simulink model "Controller_damping_cbf_22"  (R2022b)
settings: Solver=ode4  StartTime=0.0  StopTime=Inf  FixedStep=1e-3  RelTol=1e-3
values from neighbouring files (symbols this model uses):
  cbf_damping_params = [cbf_p_ths; cbf_v_ths; cbf_v_0; cbf_gamma; cbf_d_max;                        cbf_w_lin; cbf_w_quad; plane_normal; plane_offset;                        cbf_latch_entry; cbf_zone_hyst; cbf_latch_alpha; cbf_clip_drift;                        cbf_tau_rate; cbf_dt; cbf_gamma_pos_scale]    [init_damping_cbf.m]
  Dn = 20 * ones(7,1)    [init_damping_cbf.m]
  H_0_cy = H_0_pr * H_pr_cy    [init_damping_cbf.m]
  H_home = getTransform(Franka_robot, q_home, 'panda_link8', 'panda_link0')    [init_damping_cbf.m]
  Kn = 0 * ones(7,1)    [init_damping_cbf.m]
  q_home = q_init    [init_damping_cbf.m]
  q_init = [0 0  0  -(2/4)*pi  0  pi/2  -pi/4]'    [init_damping_cbf.m]
undefined symbols (not defined in the file or in its folder): DiscIntNeverNeededParam, Fext_mag, T_final, X, Y, Z
libraries: sm_lib x162, nesl_utility x44, matrix_library x3, Robotics_lib x1
(part 1 of 12)
settings Model: Creator=nthelenb  LastModifiedBy=galileo
settings ConfigComp: CovMetricSettings=de  CovBoundaryAbsTol=1.0e-5
settings SimscapeCC: SimscapeUseEnergyAccounting=off

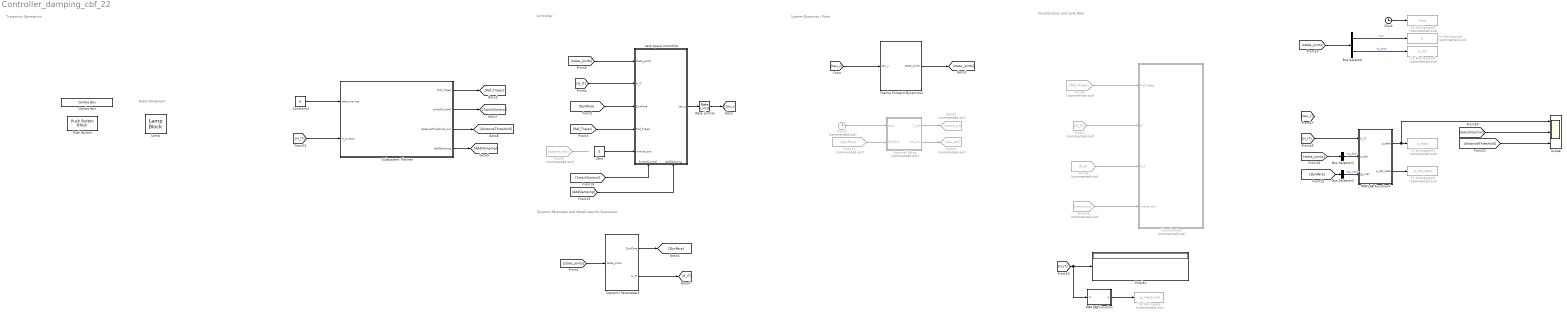
== system Controller_damping_cbf_22 ==
  note: Visualiszation and save Data
  note: Robot Movement
  note: Dynamic Parameter and Model Specific Quantities
  note: System Dynamics / Plant
  note: Trajectory Generation
  note: Controller
  Bus Selector : BusSelector  OutputSignals=q,q_dot
  Bus Selector1 : BusSelector  OutputSignals=q_dot
  Bus Selector2 : BusSelector  OutputSignals=Jg_mat
  Clock : Clock
  Clock1 : Clock  Commented=on
  Combo Box : ComboBox  LabelPosition=Hide  SelectedLabel=Move Gravi. Comp
      settings: Values={{'Go Home', 'Move Gravi. Comp', 'Move Add Damp'}, [1 2 3]}
  Constant3 : Constant  Value=0
  Display : Display
  Dynamic Parameters : Subsystem
  External Force : Subsystem  Commented=on
  Franka Forward Dynamics2 : Subsystem
  From11 : From  Commented=on  GotoTag=DynPara
  From14 : From  Commented=on  GotoTag=wrench_ext
  From5 : From  Commented=on  GotoTag=K_d
  From7 : From  Commented=on  GotoTag=H_IT
  From8 : From  Commented=on  GotoTag=Ref_Trajec
  From9 : From  Commented=on  GotoTag=wrench_ext
  Goto5 : Goto  Commented=on  GotoTag=wrench_ext
  Goto6 : Goto  Commented=on  GotoTag=tau_ext
  Lamp : LampBlock  LabelPosition=Hide
  MATLAB Function : MATLAB Function  TreatAsAtomicUnit=on
  MATLAB Function4 : MATLAB Function  TreatAsAtomicUnit=on
  Push Button : PushButtonBlock  ButtonText=Move Robot  OffValue=0.000000
  Rate Limiter : RateLimiter  RisingSlewLimit=999  FallingSlewLimit=-999  SampleTimeMode=inherited
  Scope : Scope  NumInputPorts=3
  Subsystem: Planner : Subsystem
  To Workspace : ToWorkspace  Commented=on  VariableName=p_measured  SampleTime=-1
  To Workspace3 : ToWorkspace  Commented=on  VariableName=q  SampleTime=-1
  To Workspace4 : ToWorkspace  Commented=on  VariableName=q_dot  SampleTime=-1
  To Workspace5 : ToWorkspace  Commented=on  VariableName=p_data  SampleTime=-1
  To Workspace6 : ToWorkspace  Commented=on  VariableName=p_dot_data  SampleTime=-1
  To Workspace8 : ToWorkspace  Commented=on  VariableName=time  SampleTime=-1
  Visualisation : Subsystem  Commented=on
  Zero : Constant  Value=0  OutDataTypeStr=Inherit: Inherit via back propagation
  task space controller : Subsystem
      settings: PortSchema="{\"entries\":[{\"content\":{\"sides\":[{\"content\":{\"connectorIds\":[\"In1\",\"In2\",\"In3\",\"In4\",\"In5\"]},\"type\":\"ConnectorPlacement.EquallySpacedRectSide\",\"uuid\":\"77049308-6373-4cc5-ac04-ffe2481fe586\"},{\"content\":{\"connectorIds\":[\"Out1\"],\"side\":\"RIGHT\"},\"type\":\"ConnectorPlacement.EquallySpacedRectSide\",\"uuid\":\"f03c39fe-2f04-4b7b-9f47-c34b5694c009\"},{\"content\":{\"connectorIds\":[],\"side\":\"TOP\"},\"type\":\"ConnectorPlacement.EquallySpacedRectSide\",\"uuid\":\"88522150-2a14-460b-940a-8c2ff3633826\"},{\"content\":{\"connectorIds\":[\"In6\",\"In7\"],\"side\":\"BOTTOM\"},\"type\":\"ConnectorPlacement.EquallySpacedRectSide\",\"uuid\":\"dd94313b-0570-425b-8d26-1c571736a013\"}]},\"type\":\"ConnectorPlacement.EquallySpacedConnector\",\"uuid\":\"5aa11ebf-be9b-4d28-87ba-ea9d43661d80\"}],\"packageUris\":[\"http://schema.mathworks.com/mf0/Connector/R2020b\"],\"version\":\"1.0\"}"
  wires:
  External Force/1(F_ext) -> Goto5/1
  From11/1 -> External Force/2(DynPara)
  Clock1/1 -> External Force/1(time)
  External Force/2(tau_ext) -> Goto6/1
  Franka Forward Dynamics2/1(state_joints) -> [state_joints]
  [tau_c] -> Franka Forward Dynamics2/1(tau_c)
  [state_joints] -> Dynamic Parameters/1(state_joints)
  Zero/1 -> task space controller/5(wrench_ext)
  From7/1 -> Visualisation/2(H)
  [AddDamping] -> task space controller/7(AddDamping)
  Subsystem: Planner/4(AddDamping) -> [AddDamping]
  Clock/1 -> To Workspace8/1
  Constant3/1 -> Subsystem: Planner/1(start_moving)
  Bus Selector2/1 -> MATLAB Function4/3(Jg_mat)  "<Jg_mat>"
  [distanceThreshold] -> Scope/3
  [H_IT] -> task space controller/2(H_IT)
  From9/1 -> ?
  From8/1 -> Visualisation/1(Ref_Trajec)
  [state_joints] -> task space controller/1(state_joints)
  Subsystem: Planner/3(distanceThreshold_out) -> [distanceThreshold]
  MATLAB Function4/1(p_data) -> Scope/1, To Workspace5/1
  From14/1 -> Visualisation/4(wrench_ext)
  [SwitchControl] -> Scope/2
  [DynPara] -> Bus Selector2/1
  Bus Selector/2 -> To Workspace4/1  "<q_dot>"
  [SwitchControl] -> task space controller/6(SwitchControl)
  MATLAB Function4/2(p_dot_data) -> To Workspace6/1
  Subsystem: Planner/1(Ref_Trajec) -> [Ref_Trajec]
  [state_joints] -> Bus Selector/1
  [state_joints] -> Bus Selector1/1
  Subsystem: Planner/2(switchControl) -> [SwitchControl]
  [H_IT] -> MATLAB Function4/1(H_IT)
  Rate Limiter/1 -> [tau_c]
  Bus Selector1/1 -> MATLAB Function4/2(q_dot)  "<q_dot>"
  task space controller/1(tau_c) -> Rate Limiter/1
  [H_IT] -> MATLAB Function/1(H), Display/1
  [Ref_Trajec] -> task space controller/4(Ref_Trajec)
  [DynPara] -> task space controller/3(DynPara)
  MATLAB Function/1(p) -> To Workspace/1
  Dynamic Parameters/1(DynPara) -> [DynPara]
  Bus Selector/1 -> To Workspace3/1  "<q>"
  [H_IT] -> Subsystem: Planner/2(H_current)
  From5/1 -> Visualisation/3(K_d)
  Dynamic Parameters/2(H_IT) -> [H_IT]

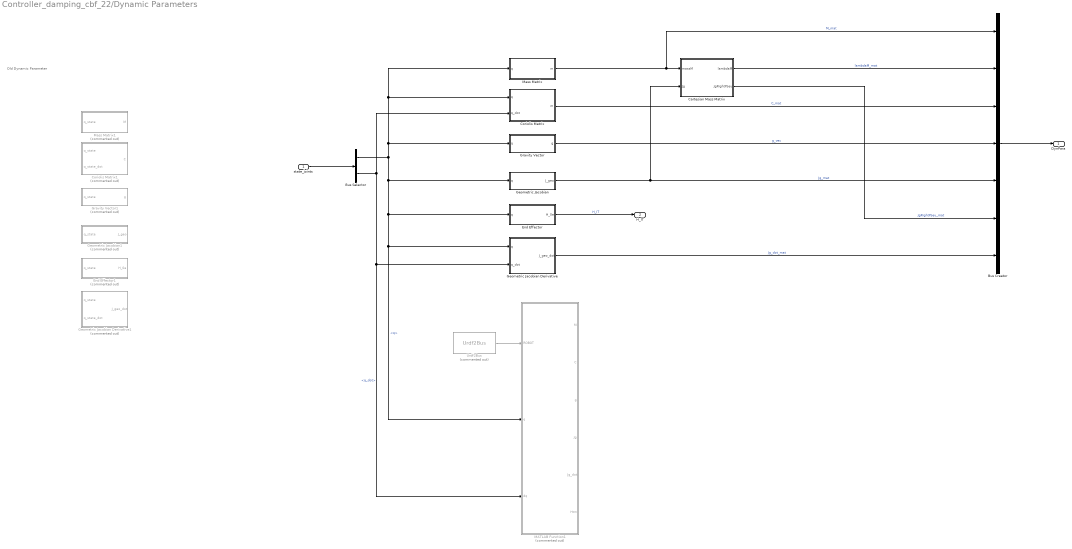
== system Controller_damping_cbf_22/Dynamic Parameters ==
  note: Old Dynamic Parameter
  state_joints : Inport
  Bus Creator : BusCreator  Inputs=7
  Bus Selector : BusSelector  OutputSignals=q,q_dot
  Cartesian Mass Matrix : MATLAB Function  TreatAsAtomicUnit=on
  Coriolis Matrix : MATLAB Function  TreatAsAtomicUnit=on
  Coriolis Matrix1 : MATLAB Function  Commented=on  TreatAsAtomicUnit=on
  End Effector : MATLAB Function  TreatAsAtomicUnit=on
  End Effector1 : MATLAB Function  Commented=on  TreatAsAtomicUnit=on
  Geometric Jacobian : MATLAB Function  TreatAsAtomicUnit=on
  Geometric Jacobian Derivative : MATLAB Function  TreatAsAtomicUnit=on
  Geometric Jacobian Derivative1 : MATLAB Function  Commented=on  TreatAsAtomicUnit=on
  Geometric Jacobian1 : MATLAB Function  Commented=on  TreatAsAtomicUnit=on
  Gravity Vector : MATLAB Function  TreatAsAtomicUnit=on
  Gravity Vector1 : MATLAB Function  Commented=on  TreatAsAtomicUnit=on
  MATLAB Function1 : MATLAB Function  Commented=on  TreatAsAtomicUnit=on
  Mass Matrix : MATLAB Function  TreatAsAtomicUnit=on
  Mass Matrix1 : MATLAB Function  Commented=on  TreatAsAtomicUnit=on
  Urdf2Bus : Robotics_lib/Urdf2Bus  Commented=on  filename='Franka_arm.urdf'  tcp=9  S=[]
  DynPara : Outport
  H_IT : Outport  Port=2
  wires:
  state_joints/1 -> Bus Selector/1
  Urdf2Bus/1 -> MATLAB Function1/1(ROBOT)
  Bus Selector/1 -> Coriolis Matrix/1(q), Mass Matrix/1(q), Gravity Vector/1(q), Geometric Jacobian/1(q), MATLAB Function1/2(q), Geometric Jacobian Derivative/1(q), End Effector/1(q)  "<q>"
  Bus Selector/2 -> Geometric Jacobian Derivative/2(q_dot), MATLAB Function1/3(dq), Coriolis Matrix/2(q_dot)  "<q_dot>"
  Mass Matrix/1(m) -> Bus Creator/1, Cartesian Mass Matrix/1(massM)  "M_mat"
  Bus Creator/1 -> DynPara/1
  Cartesian Mass Matrix/1(lambdaM) -> Bus Creator/2  "lambdaM_mat"
  Coriolis Matrix/1(m) -> Bus Creator/3  "C_mat"
  Gravity Vector/1(g) -> Bus Creator/4  "g_vec"
  Cartesian Mass Matrix/2(JgRightPseu) -> Bus Creator/6  "JgRightPseu_mat"
  Geometric Jacobian Derivative/1(J_geo_dot) -> Bus Creator/7  "Jg_dot_mat"
  End Effector/1(H_0e) -> H_IT/1  "H_IT"
  Geometric Jacobian/1(J_geo) -> Cartesian Mass Matrix/2(Jg), Bus Creator/5  "Jg_mat"

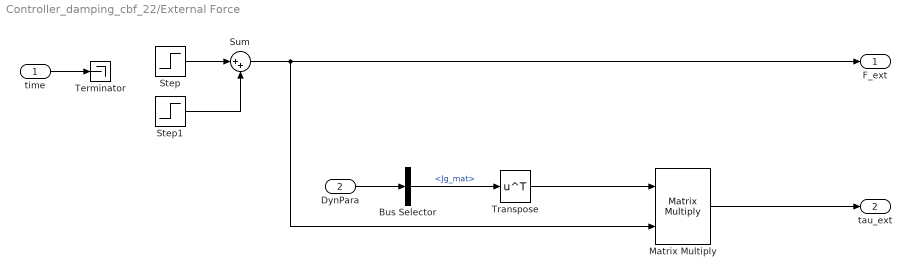
== system Controller_damping_cbf_22/External Force ==
  time : Inport
  DynPara : Inport  Port=2
  Bus Selector : BusSelector  OutputSignals=Jg_mat
  Matrix Multiply : Product  Multiplication=Matrix(*)
  Step : Step  Time=5  Before=zeros(6,1)  After=Fext_mag.*[1;zeros(5,1)]  SampleTime=0
  Step1 : Step  Time=12  Before=zeros(6,1)  After=-Fext_mag.*[1;zeros(5,1)]  SampleTime=0
  Sum : Sum  Inputs=|++
  Terminator : Terminator
  Transpose : Math  Operator=transpose
  F_ext : Outport
  tau_ext : Outport  Port=2
  wires:
  Step/1 -> Sum/1
  Step1/1 -> Sum/2
  time/1 -> Terminator/1
  Sum/1 -> Matrix Multiply/2, F_ext/1
  Transpose/1 -> Matrix Multiply/1
  Bus Selector/1 -> Transpose/1  "<Jg_mat>"
  DynPara/1 -> Bus Selector/1
  Matrix Multiply/1 -> tau_ext/1

== system Controller_damping_cbf_22/Franka Forward Dynamics2 ==
  note: NO joint Limits
  note: With joint Limits
  tau_c : Inport
  Bus Creator : BusCreator  Inputs=2
  Franka Forward Dynamics [SimMechanics] : Subsystem
  Franka Forward Dynamics [SimMechanics]1 : Subsystem  Commented=on
  state_joints : Outport
  wires:
  Franka Forward Dynamics [SimMechanics]/1(q) -> Bus Creator/1  "q"
  Franka Forward Dynamics [SimMechanics]/2(q_dot) -> Bus Creator/2  "q_dot"
  tau_c/1 -> Franka Forward Dynamics [SimMechanics]/1(tau)
  Bus Creator/1 -> state_joints/1

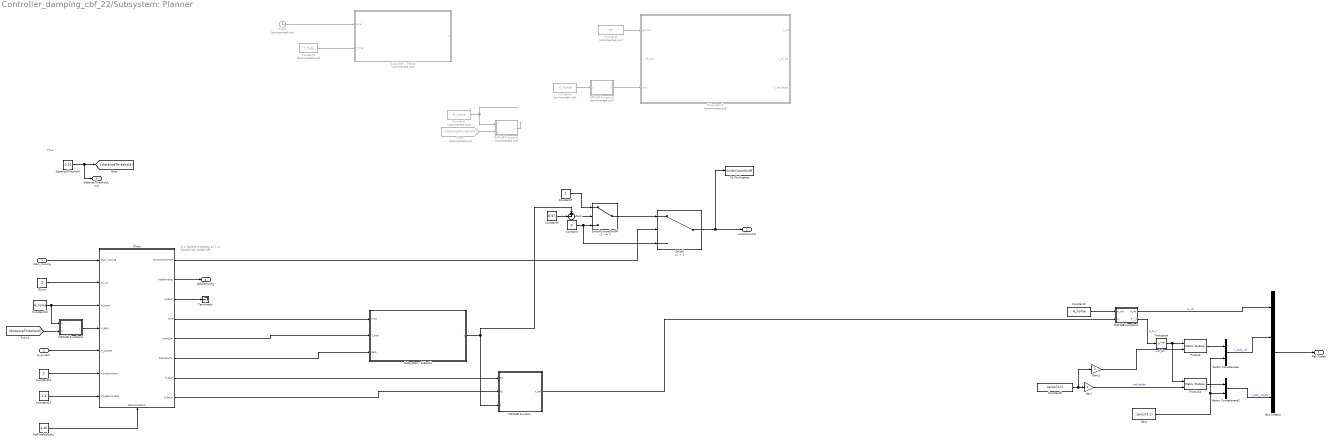
== system Controller_damping_cbf_22/Subsystem: Planner ==
  note: 0 = Control is always on
      | 1 = Control can switch off
  note: Para
  start_moving : Inport
  H_current : Inport  Port=2
  Bus Creator : BusCreator  Inputs=4
  Chart : Stateflow chart  TreatAsAtomicUnit=on
      settings: PortSchema="{\"entries\":[{\"content\":{\"sides\":[{\"content\":{\"connectorIds\":[\"In2\",\"In3\",\"In5\",\"In4\",\"In6\",\"In7\",\"In8\"]},\"type\":\"ConnectorPlacement.EquallySpacedRectSide\",\"uuid\":\"9d0e544c-68a3-4d0d-81a9-b4a9e24909b9\"},{\"content\":{\"connectorIds\":[\"Out1\",\"Out2\",\"Out4\",\"Out5\",\"Out3\",\"Out6\",\"Out7\",\"Out8\"],\"side\":\"RIGHT\"},\"type\":\"ConnectorPlacement.EquallySpacedRectSide\",\"uuid\":\"6b3881b7-7b6b-4877-af69-7085981ee4af\"},{\"content\":{\"connectorIds\":[],\"side\":\"TOP\"},\"type\":\"ConnectorPlacement.EquallySpacedRectSide\",\"uuid\":\"e07b297f-72d7-4e07-a8ff-78e8d5f0a2d3\"},{\"content\":{\"connectorIds\":[\"In1\"],\"side\":\"BOTTOM\"},\"type\":\"ConnectorPlacement.EquallySpacedRectSide\",\"uuid\":\"0f8bb3c0-13a8-44a0-b297-dd122208e0f5\"}]},\"type\":\"ConnectorPlacement.EquallySpacedConnector\",\"uuid\":\"f28dcff5-d9f4-4a6b-99a1-2f2896a9f903\"}],\"packageUris\":[\"http://schema.mathworks.com/mf0/Connector/R2020b\"],\"version\":\"1.0\"}"
  Clock : Clock  Commented=on
  Constant : Constant  Value=0
  Constant1 : Constant  Commented=on  Value=H_home
  Constant10 : Constant  Value=H_home
  Constant11 : Constant  Value=1.4
  Constant12 : Constant  Value=3
  Constant2 : Constant  Value=H_home
  Constant3 : Constant  Commented=on  Value=60
  Constant4 : Constant  Commented=on  Value=T_final
  Constant5 : Constant  Commented=on  Value=H_home
  Constant6 : Constant  Value=0.97
  Constant7 : Constant
  Constant8 : Constant  Value=zeros(3,1)
  From : From  Commented=on  GotoTag=distanceThreshold
  Gain : Gain
  Gain1 : Gain
  ID_run : Constant  Value=2
  MATLAB Function : MATLAB Function  TreatAsAtomicUnit=on
  MATLAB Function1 : MATLAB Function  Commented=on  TreatAsAtomicUnit=on
  MATLAB Function2 : MATLAB Function  TreatAsAtomicUnit=on
  MATLAB Function3 : MATLAB Function  Commented=on  TreatAsAtomicUnit=on
  MATLAB Function4 : MATLAB Function  TreatAsAtomicUnit=on
  Product : Product  Multiplication=Matrix(*)
  Product3 : Product  Multiplication=Matrix(*)
  SetFinalVelocity : Constant  Value=2.45
  Subsystem2 : Subsystem  Commented=on
  Subsystem: S-Block : Subsystem  Commented=on
  Subsystem: S-Block1 : Subsystem
  Sum : Sum  Inputs=+-|
  Switch : Switch  Criteria=u2 > Threshold  SaturateOnIntegerOverflow=off  InputSameDT=off
  SwitchControlOnOff : Switch  SaturateOnIntegerOverflow=off  InputSameDT=off
  Terminator : Terminator
  To Workspace : ToWorkspace  VariableName=SwitchControlOnOff  SampleTime=-1
  Transpose : Math  Operator=transpose
  Vector Concatenate : Concatenate
  Vector Concatenate2 : Concatenate
  Zero : Constant  Value=zeros(3,1)  OutDataTypeStr=Inherit: Inherit via back propagation
  distanceThreshold : Constant  Value=0.31
  Ref_Trajec : Outport
  switchControl : Outport  Port=2
  distanceThreshold_out : Outport  Port=3
  AddDamping : Outport  Port=4
  wires:
  Zero/1 -> Vector Concatenate/2, Vector Concatenate2/2
  Product/1 -> Vector Concatenate/1
  Bus Creator/1 -> Ref_Trajec/1
  Vector Concatenate2/1 -> Bus Creator/4  "V_body_ref_dot"
  MATLAB Function2/2(R_I_t) -> Transpose/1  "R_ts_t"
  MATLAB Function2/1(H_ref) -> Bus Creator/1  "H_ref"
  Clock/1 -> Subsystem: S-Block/1(time)
  Constant2/1 -> MATLAB Function2/1(H_init)
  Constant4/1 -> Subsystem: S-Block/2(T_final)
  Gain1/1 -> Product/2  "xref_dot"
  Product3/1 -> Vector Concatenate2/1
  Subsystem: S-Block1/1(s) -> Sum/1, MATLAB Function/3(s)
  Transpose/1 -> Product3/1, Product/1
  Vector Concatenate/1 -> Bus Creator/2  "V_body_ref"
  Gain/1 -> Product3/2  "xref_dotdot"
  MATLAB Function1/1(y) -> ?
  Constant1/1 -> MATLAB Function1/1(H)
  MATLAB Function/1(x_ref) -> MATLAB Function2/2(d)
  Constant3/1 -> Subsystem2/1(gamma)
  Constant5/1 -> MATLAB Function3/1(u)
  MATLAB Function3/1(y) -> Subsystem2/3(xInit)
  From/1 -> MATLAB Function1/2(z)
  distanceThreshold/1 -> distanceThreshold_out/1, [distanceThreshold]
  Constant/1 -> Switch/3, SwitchControlOnOff/3
  SwitchControlOnOff/1 -> Switch/1
  Sum/1 -> SwitchControlOnOff/2
  Constant6/1 -> Sum/2
  Constant7/1 -> SwitchControlOnOff/1
  Constant8/1 -> Gain1/1, Gain/1
  Chart/5(time) -> Subsystem: S-Block1/1(time)
  Chart/3(moveDur) -> Subsystem: S-Block1/2(T_final)
  Chart/4(runBool) -> Terminator/1
  H_current/1 -> Chart/6(H_current)
  ID_run/1 -> Chart/3(ID_run)
  Constant11/1 -> Chart/8(moveDurImpact)
  Constant12/1 -> Chart/7(moveDurHome)
  Chart/6(finalVelocity) -> Subsystem: S-Block1/3(data)
  Chart/7(H_start) -> MATLAB Function/1(H1)
  Chart/8(H_finish) -> MATLAB Function/2(H2)
  Constant10/1 -> Chart/5(H_home), MATLAB Function4/1(H)
  [distanceThreshold] -> MATLAB Function4/2(z)
  MATLAB Function4/1(y) -> Chart/4(H_goal)
  Switch/1 -> To Workspace/1, switchControl/1
  Chart/1(TurnControlOnOff) -> Switch/2
  Chart/2(AddDamping) -> AddDamping/1
  start_moving/1 -> Chart/2(start_moving)
  SetFinalVelocity/1 -> Chart/1(SetFinalVelocity)

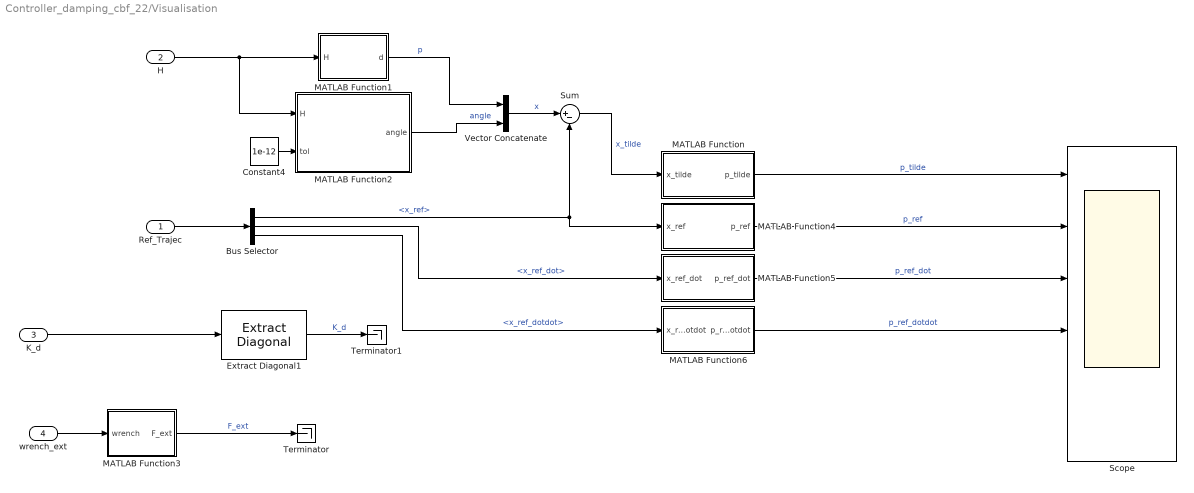
== system Controller_damping_cbf_22/Visualisation ==
  Ref_Trajec : Inport
  H : Inport  Port=2
  K_d : Inport  Port=3
  wrench_ext : Inport  Port=4
  Bus Selector : BusSelector  OutputSignals=x_ref,x_ref_dot,x_ref_dotdot
  Constant4 : Constant  Value=1e-12
  Extract Diagonal1 : matrix_library/Extract Diagonal
      settings: LibrarySourceBlock=|
      | simulink/Matrix
      | Operations/Extract Diagonal
  MATLAB Function : MATLAB Function  TreatAsAtomicUnit=on
  MATLAB Function1 : MATLAB Function  TreatAsAtomicUnit=on
  MATLAB Function2 : MATLAB Function  TreatAsAtomicUnit=on
  MATLAB Function3 : MATLAB Function  TreatAsAtomicUnit=on
  MATLAB Function4 : MATLAB Function  TreatAsAtomicUnit=on
  MATLAB Function5 : MATLAB Function  TreatAsAtomicUnit=on
  MATLAB Function6 : MATLAB Function  TreatAsAtomicUnit=on
  Scope : Scope  NumInputPorts=6
  Sum : Sum  Inputs=|+-
  Terminator : Terminator
  Terminator1 : Terminator
  Vector Concatenate : Concatenate
  wires:
  H/1 -> MATLAB Function2/1(H), MATLAB Function1/1(H)
  MATLAB Function1/1(d) -> Vector Concatenate/1  "p"
  Ref_Trajec/1 -> Bus Selector/1
  Bus Selector/1 -> MATLAB Function4/1(x_ref), Sum/2  "<x_ref>"
  MATLAB Function/1(p_tilde) -> Scope/1  "p_tilde"
  Constant4/1 -> MATLAB Function2/2(tol)
  MATLAB Function2/1(angle) -> Vector Concatenate/2  "angle"
  Vector Concatenate/1 -> Sum/1  "x"
  Sum/1 -> MATLAB Function/1(x_tilde)  "x_tilde"
  Extract Diagonal1/1 -> Terminator1/1  "K_d"
  wrench_ext/1 -> MATLAB Function3/1(wrench)
  MATLAB Function3/1(F_ext) -> Terminator/1  "F_ext"
  K_d/1 -> Extract Diagonal1/1
  MATLAB Function4/1(p_ref) -> Scope/2  "p_ref"
  MATLAB Function5/1(p_ref_dot) -> Scope/3  "p_ref_dot"
  Bus Selector/2 -> MATLAB Function5/1(x_ref_dot)  "<x_ref_dot>"
  MATLAB Function6/1(p_ref_dotdot) -> Scope/4  "p_ref_dotdot"
  Bus Selector/3 -> MATLAB Function6/1(x_ref_dotdot)  "<x_ref_dotdot>"

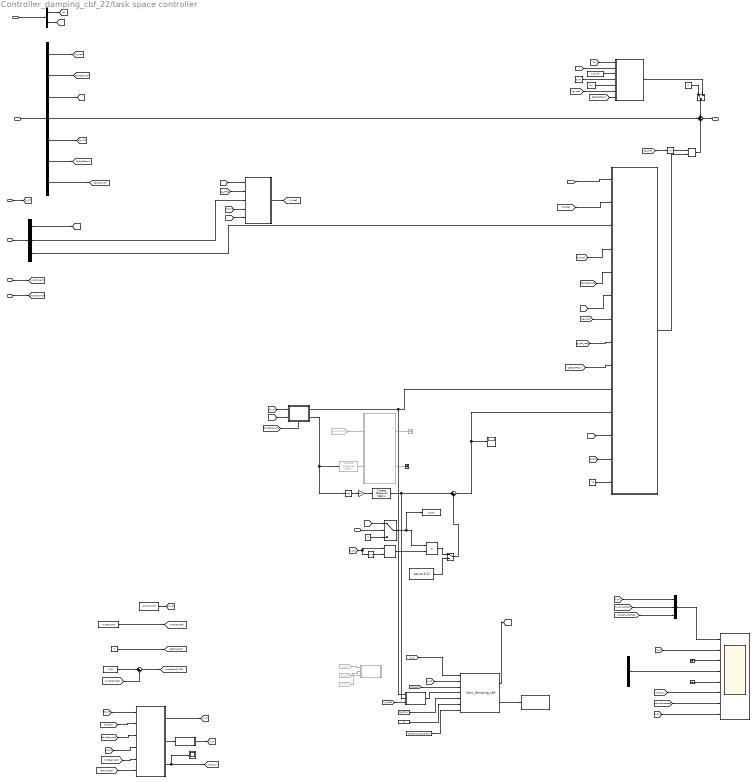
== system Controller_damping_cbf_22/task space controller ==
  note: normalvector of hyperplane
      | + 3 zeros for the angular part
  note: with Box set = 0.106 m
      | regular table without box set = -0.004
      | Box on Table = 0.106-0.004
  note: with Waping endeffector set = 0.055
  note: (1 - x/x0)^expo
  note: 0 = constant
      | 1 = Christian's
      | 2 = My first
      | 3 = General Function
  note: Alt: -2e-3
      | Versuch: -5e-3
  note: 0 = org
      | 1 = moduled
  note: Visualisation
  state_joints : Inport
  H_IT : Inport  Port=2
  DynPara : Inport  Port=3
  Ref_Trajec : Inport  Port=4
  wrench_ext : Inport  Port=5
  SwitchControl : Inport  Port=6
  AddDamping : Inport  Port=7
  Additional_Damping : Constant  Value=70
  Bus Selector : BusSelector  OutputSignals=H_ref,V_body_ref,V_body_ref_dot
  Bus Selector1 : BusSelector  OutputSignals=q,q_dot
  Bus Selector2 : BusSelector  OutputSignals=M_mat,lambdaM_mat,C_mat,g_vec,Jg_mat,JgRightPseu_mat,Jg_dot_mat
  CBF_Telemetry_Visualizer : Subsystem
  Compute_F_nominal : MATLAB Function  TreatAsAtomicUnit=on
  Compute_vc_ground : MATLAB Function  Commented=on  TreatAsAtomicUnit=on
  Constant : Constant  Value=Dn
  Constant10 : Constant  Value=zeros(6,6)
  Constant3 : Constant  Value=q_home
  Constant4 : Constant  Value=0.*Kn
  Constant7 : Constant  Value=[0;0;1;0;0;0]  VectorParams1D=off
  Constant8 : Constant  Value=0
  Constant_Fext_damp : Constant  Value=zeros(6,1)
  Constant_cbf_params : Constant  Value=cbf_damping_params
  Constant_use_fext_damp : Constant  Value=0
  Create Diagonal Matrix : matrix_library/Create Diagonal Matrix  Commented=on
      settings: LibrarySourceBlock=|
      | simulink/Matrix
      | Operations/Create Diagonal
      | Matrix
  Create Diagonal Matrix1 : matrix_library/Create Diagonal Matrix
      settings: LibrarySourceBlock=|
      | simulink/Matrix
      | Operations/Create Diagonal
      | Matrix
  Damping Desing Selection : Subsystem  Commented=on
  Display : Display
  From1 : From  Commented=on  GotoTag=lambda_mat
  From_Jg_damp : From  Commented=on  GotoTag=Jg_mat
  From_nhp_damp : From  Commented=on  GotoTag=n_hp
  From_qdot_damp : From  Commented=on  GotoTag=q_dot
  Gain : Gain  Gain=0.6
  Ground_Scope_3 : Ground
  Ground_Scope_5 : Ground
  MATLAB Function2 : MATLAB Function  TreatAsAtomicUnit=on
  Manual Switch : ManualSwitch
  Manual Switch1 : ManualSwitch
  MatrixMultiply1 : Product  Multiplication=Matrix(*)
  MatrixMultiply2 : Product  Multiplication=Matrix(*)
  MatrixMultiply3 : Product
  S-Function Damping CBF : S-Function  FunctionName=sfun_damping_cbf  SFunctionDeploymentMode=off  EnableBusSupport=off
  Scope3 : Scope
  Scope:DapingPara1 : Scope  NumInputPorts=8
  Sqrt : Sqrt
  Stiffnessforces : Subsystem
      settings: PortSchema="{\"entries\":[{\"content\":{\"sides\":[{\"content\":{\"connectorIds\":[\"In1\",\"In2\"]},\"type\":\"ConnectorPlacement.EquallySpacedRectSide\",\"uuid\":\"1468fc71-913f-41d6-90e8-02e3f9f938f0\"},{\"content\":{\"connectorIds\":[\"Out1\",\"Out2\"],\"side\":\"RIGHT\"},\"type\":\"ConnectorPlacement.EquallySpacedRectSide\",\"uuid\":\"95c6e15f-ef93-4b77-ba6a-3736a5b46450\"},{\"content\":{\"connectorIds\":[],\"side\":\"TOP\"},\"type\":\"ConnectorPlacement.EquallySpacedRectSide\",\"uuid\":\"2bc5a35a-7ecf-444d-a182-7037bf7c7fcb\"},{\"content\":{\"connectorIds\":[\"In3\"],\"side\":\"BOTTOM\"},\"type\":\"ConnectorPlacement.EquallySpacedRectSide\",\"uuid\":\"7a866046-04ea-43c9-aace-e539a58eed94\"}]},\"type\":\"ConnectorPlacement.EquallySpacedConnector\",\"uuid\":\"cbc65bc5-8091-424d-a820-445173990e50\"}],\"packageUris\":[\"http://schema.mathworks.com/mf0/Connector/R2020b\"],\"version\":\"1.0\"}"
  Subsystem2 : Subsystem
  Subsystem4 : Subsystem
  Sum : Sum  Inputs=+++
  Sum3 : Sum  Inputs=|++
  Sum4 : Sum  Inputs=|+-
  Switch2 : Switch  Criteria=u2 > Threshold  SaturateOnIntegerOverflow=off  InputSameDT=off
  Terminator : Terminator
  Terminator2 : Terminator  Commented=on
  To Workspace : ToWorkspace  VariableName=d_add  SampleTime=-1
  Transpose : Math  Operator=transpose
  Transpose1 : Math  Operator=transpose
  Vector Concatenate2 : Concatenate  NumInputs=3
  Vector Concatenate3 : Concatenate  NumInputs=1
  Zero : Constant  Value=0  OutDataTypeStr=Inherit: Inherit via back propagation
  endEffector_height : Constant  Value=0
  impedance controller1 : MATLAB Function  TreatAsAtomicUnit=on
  nullspace damping : MATLAB Function  TreatAsAtomicUnit=on
  xTableHight : Constant  Value=0.106-0.004
  xthreshold_TSD : Constant  Value=0.30
  tau_c : Outport
  wires:
  state_joints/1 -> Bus Selector1/1
  Sum/1 -> tau_c/1
  Constant/1 -> nullspace damping/5(Dn)
  Bus Selector/1 -> [H_ref]  "<H_ref>"
  Bus Selector/2 -> Subsystem4/3(V_body_ref)  "<V_body_ref>"
  MatrixMultiply1/1 -> Sum/3
  nullspace damping/1(tau_nullspace) -> Manual Switch/2  "tau_null"
  Ref_Trajec/1 -> Bus Selector/1
  Bus Selector/3 -> impedance controller1/3(V_ref_dot)  "<V_body_ref_dot>"
  DynPara/1 -> Bus Selector2/1
  Bus Selector2/1 -> [M_mat]  "<M_mat>"
  Bus Selector2/3 -> [C_mat]  "<C_mat>"
  Bus Selector2/4 -> Sum/2  "<g_vec>"
  [q] -> nullspace damping/1(q)
  Bus Selector2/5 -> [Jg_mat]  "<Jg_mat>"
  Bus Selector2/7 -> [Jg_dot_mat]  "<Jg_dot_mat>"
  [Jg_mat] -> nullspace damping/6(Jg)
  Bus Selector2/2 -> [lambda_mat]  "<lambdaM_mat>"
  Constant3/1 -> nullspace damping/3(q_ref)
  Constant4/1 -> nullspace damping/4(Kn)
  Bus Selector2/6 -> [JgRightPseu]  "<JgRightPseu_mat>"
  [JgRightPseu] -> nullspace damping/7(JgRightPseu)
  Bus Selector1/2 -> [q_dot]  "<q_dot>"
  [q_dot] -> nullspace damping/2(q_dot)
  [q_dot] -> impedance controller1/1(q_dot)
  From1/1 -> Damping Desing Selection/1(Lambda_mat)
  Bus Selector1/1 -> [q]  "<q>"
  wrench_ext/1 -> [wrench_ext]
  Zero/1 -> Manual Switch/1
  Create Diagonal Matrix/1 -> Damping Desing Selection/2(Kd)
  Sum3/1 -> impedance controller1/11(Dd), Display/1
  xthreshold_TSD/1 -> Sum4/1
  [V_tilde] -> MATLAB Function2/2(V_tilde)
  [H_IT] -> MATLAB Function2/1(H_IT)
  [lambda_mat] -> MATLAB Function2/3(lambda_mat)
  xTableHight/1 -> [xTableHight]
  MATLAB Function2/1(x_c) -> [x_c]
  Subsystem2/1(x) -> [v_c]  "v_c"
  [q_dot] -> Subsystem4/1(q_dot)
  [Jg_mat] -> Subsystem4/2(Jg)
  Subsystem4/1(V_tilde) -> [V_tilde]
  [V_tilde] -> impedance controller1/2(V_tilde)
  [M_mat] -> impedance controller1/4(massM)
  [lambda_mat] -> impedance controller1/5(lambdaM)
  [C_mat] -> impedance controller1/6(C)
  [Jg_mat] -> impedance controller1/7(Jg)
  [Jg_dot_mat] -> impedance controller1/8(Jg_dot)
  [JgRightPseu] -> impedance controller1/9(JgRightPseu)
  Stiffnessforces/1(Fk) -> impedance controller1/10(Fk), Compute_F_nominal/1(Fk)
  [H_ref] -> Subsystem4/5(H_ref)
  [H_ref] -> Stiffnessforces/2(H_ref)
  [H_ref] -> impedance controller1/12(H_I_D)
  Stiffnessforces/2(K_d) -> Create Diagonal Matrix/1, Sqrt/1
  H_IT/1 -> [H_IT]
  [H_IT] -> Subsystem4/4(Htm)
  [H_IT] -> Stiffnessforces/1(H)
  Damping Desing Selection/1(K_ref) -> Terminator2/1
  Manual Switch/1 -> Sum/1
  endEffector_height/1 -> [eef_height]
  Constant7/1 -> [n_hp]
  MATLAB Function2/3(m_c) -> Scope3/1, [mass_c]
  [n_hp] -> MATLAB Function2/4(n_hp)
  [n_hp] -> impedance controller1/13(n_hp)
  Additional_Damping/1 -> impedance controller1/14(d_add)
  impedance controller1/1(F_control) -> MatrixMultiply1/2
  [Jg_mat] -> Transpose/1
  Transpose/1 -> MatrixMultiply1/1
  [n_hp] -> MatrixMultiply2/1, Transpose1/1
  Transpose1/1 -> MatrixMultiply2/2
  MatrixMultiply2/1 -> MatrixMultiply3/2
  Switch2/1 -> To Workspace/1, MatrixMultiply3/1
  Sqrt/1 -> Gain/1
  Gain/1 -> Create Diagonal Matrix1/1
  Create Diagonal Matrix1/1 -> Sum3/1, Compute_F_nominal/2(D0)
  [xTableHight] -> MATLAB Function2/5(xTableHight)
  [eef_height] -> MATLAB Function2/6(eef_height)
  SwitchControl/1 -> [SwitchControl]
  [SwitchControl] -> Stiffnessforces/3(SwitchControl)
  [xTableHight] -> Sum4/2
  Sum4/1 -> [xthreshold_TSD]
  Manual Switch1/1 -> Sum3/2
  [damp] -> Switch2/1
  Constant8/1 -> Switch2/3
  AddDamping/1 -> Switch2/2
  MATLAB Function2/2(v_c) -> Subsystem2/1(u)  "v_c"
  [x_c] -> Vector Concatenate2/1  "x_c"
  [xthreshold_TSD] -> Vector Concatenate2/3  "xthreshold_TSD"
  Vector Concatenate3/1 -> Scope:DapingPara1/4
  [pointOfIntersec] -> Scope:DapingPara1/7  "pointOfIntersec"
  [x_c_modified] -> Vector Concatenate2/2  "x_c_modified"
  [n_hp] -> Scope:DapingPara1/8  "n_hp"
  Vector Concatenate2/1 -> Scope:DapingPara1/1
  [mass_c] -> Scope:DapingPara1/6
  [v_c] -> Scope:DapingPara1/2  "v_c"
  Damping Desing Selection/2(D_ref) -> Terminator/1
  Constant10/1 -> Manual Switch1/2
  MatrixMultiply3/1 -> Manual Switch1/1
  Ground_Scope_3/1 -> Scope:DapingPara1/3
  Ground_Scope_5/1 -> Scope:DapingPara1/5
  From_nhp_damp/1 -> Compute_vc_ground/1(n_hp)
  From_Jg_damp/1 -> Compute_vc_ground/2(Jg)
  From_qdot_damp/1 -> Compute_vc_ground/3(q_dot)
  [V_tilde] -> Compute_F_nominal/3(V_tilde)
  [x_c] -> S-Function Damping CBF/1
  [mass_c] -> S-Function Damping CBF/3
  Compute_F_nominal/1(F_nominal) -> S-Function Damping CBF/4
  Constant_Fext_damp/1 -> S-Function Damping CBF/5
  Constant_use_fext_damp/1 -> S-Function Damping CBF/6
  Constant_cbf_params/1 -> S-Function Damping CBF/7
  S-Function Damping CBF/1 -> [damp]
  S-Function Damping CBF/2 -> CBF_Telemetry_Visualizer/1(telem)
  [v_c] -> S-Function Damping CBF/2

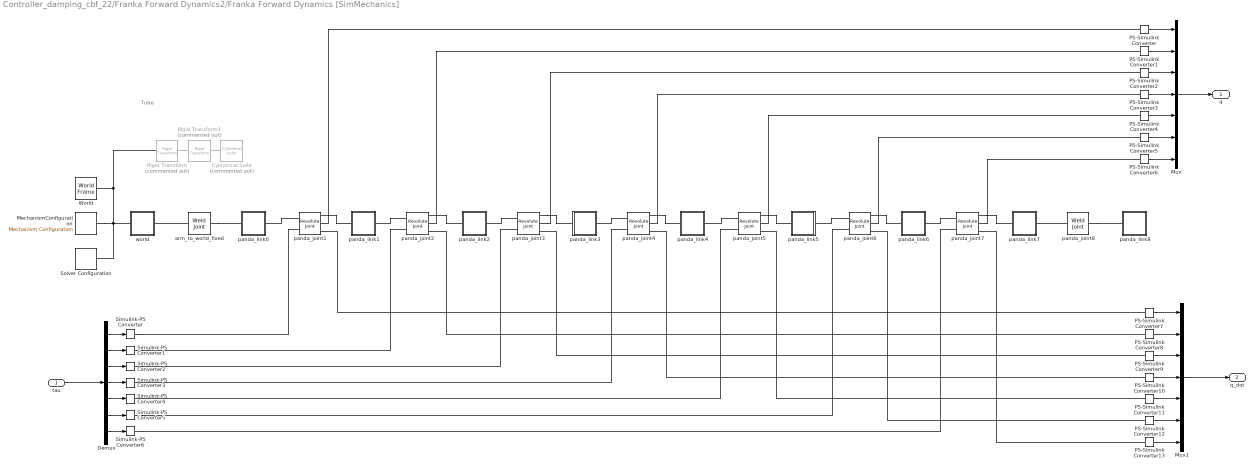
== system Controller_damping_cbf_22/Franka Forward Dynamics2/Franka Forward Dynamics [SimMechanics] ==
  note: Tube
  tau : Inport
  Cylindrical Solid : sm_lib/Body Elements/Cylindrical Solid  Commented=on  CylinderRadius=0.13  CylinderRadiusUnits=m  CylinderLength=0.446  CylinderLengthUnits=m  ExportEntireGeometry=off  InertiaType=CalculateFromGeometry  BasedOnType=Density  Density=1000  DensityUnits=kg/m^3  Mass=1  MassUnits=kg  CenterOfMass=[0 0 0]  CenterOfMassUnits=m  MomentsOfInertia=[1 1 1]  MomentsOfInertiaUnits=kg*m^2  ProductsOfInertia=[0 0 0]  ProductsOfInertiaUnits=kg*m^2  GraphicType=FromGeometry  MarkerShape=Sphere  MarkerSize=10  GraphicVisPropType=SimpleVisualProperties  GraphicDiffuseColor=[1.0 0.0 1.0]  GraphicOpacity=1.0  GraphicSpecularColor=[0.5 0.5 0.5 1.0]  GraphicAmbientColor=[0.15 0.15 0.15 1.0]  GraphicEmissiveColor=[0.0 0.0 0.0 1.0]  GraphicShininess=75  DoExposeReferenceFrame=on  SerializedFrames=<Frames/>
  Demux : Demux  Outputs=7
  MechanismConfiguration : sm_lib/Utilities/Mechanism Configuration  UniformGravity=Constant  GravityVector=Franka_robot.Gravity  GravityVectorUnits=m/s^2  LinearizationDelta=0.001  JointModeTransitionNonlinearIterations=2
  Mux : Mux  Inputs=7
  Mux1 : Mux  Inputs=7
  PS-Simulink Converter{,1..13} (14 alike) : nesl_utility/PS-Simulink Converter  PhysicalDomain=network_engine_domain  SubClassName=ps_output  LeftPortType=input  RightPortType=output  PseudoPeriodic=off  Frequencies=[]  VectorFormat=inherit  Unit=inherit  AffineConversion=off
  Rigid Transform : sm_lib/Frames and Transforms/Rigid Transform  Commented=on  RotationMethod=RotationMatrix  FollAlignAxisA=+X  BaseAlignAxisA=+Y  FollAlignAxisB=+Y  BaseAlignAxisB=+Z  RotationStandardAxis=+Z  RotationAngle=0.0  RotationAngleUnits=deg  RotationArbitraryAxis=[0 0 1]  RotationSequenceAxes=FollowerAxes  RotationSequence=XYX  RotationSequenceAngles=[0 0 0]  RotationSequenceAnglesUnits=deg  RotationMatrix=H_0_cy(1:3,1:3)  Quaternion=[1 0 0 0]  TranslationMethod=Cartesian  TranslationCartesianOffset=H_0_cy(1:3,4)  TranslationCartesianOffsetUnits=m  TranslationStandardAxis=+Z  TranslationStandardOffset=0  TranslationStandardOffsetUnits=m  TranslationROffset=0  TranslationROffsetUnits=m  TranslationThetaOffset=0  TranslationThetaOffsetUnits=deg  TranslationZOffset=0  TranslationZOffsetUnits=m
  Rigid Transform1 : sm_lib/Frames and Transforms/Rigid Transform  Commented=on  RotationMethod=RotationMatrix  FollAlignAxisA=+X  BaseAlignAxisA=+Y  FollAlignAxisB=+Y  BaseAlignAxisB=+Z  RotationStandardAxis=+Z  RotationAngle=0.0  RotationAngleUnits=deg  RotationArbitraryAxis=[0 0 1]  RotationSequenceAxes=FollowerAxes  RotationSequence=XYX  RotationSequenceAngles=[0 0 0]  RotationSequenceAnglesUnits=deg  RotationMatrix=[0,0,1; 0,1,0; -1,0,0]  Quaternion=[1 0 0 0]  TranslationMethod=None  TranslationCartesianOffset=zeros()  TranslationCartesianOffsetUnits=m  TranslationStandardAxis=+Z  TranslationStandardOffset=0  TranslationStandardOffsetUnits=m  TranslationROffset=0  TranslationROffsetUnits=m  TranslationThetaOffset=0  TranslationThetaOffsetUnits=deg  TranslationZOffset=0  TranslationZOffsetUnits=m
  Simulink-PS Converter{,1..6} (7 alike) : nesl_utility/Simulink-PS Converter  PhysicalDomain=network_engine_domain  SubClassName=ps_input  LeftPortType=input  RightPortType=output  PseudoPeriodic=off  Frequencies=[]  NoiseDistribution=none  NoiseParameters=[]  Unit=1  AffineConversion=off  FilteringAndDerivatives=provide  SimscapeFilterOrder=1  InputFilterTimeConstant=0.001  UdotUserProvided=0
  Solver Configuration : nesl_utility/Solver Configuration  PhysicalDomain=network_engine_domain  SubClassName=solver  LeftPortType=input  RightPortType=generic  Tones=[]  Harmonics=[]  SimulateNoise=off  Profile=off  UseLocalSampling=off  EnableSwitchedLinearOptims=on  FrequencyDomain=off  UseCCode=off  RelTol=0.001  AbsTol=0.001  MinStep=1e-09  ToWorkspace=off  RevertToSquareIcSolve=off  NumHomotopyIterations=100  PhasorMode=off  PhasorModeNumHarmonics=1  ConsistencySolver=NEWTON_XTOL_AFTER_FTOL  CanonicalOrdering=UNORDERED  OptimizeIntermediates=UNOPTIMIZED  MulticoreSolverChoice=BACKWARD_EULER  IndexReductionMethod=DerivativeReplacement  DoDC=off  ResidualTolerance=1e-09  ConsistencyTolSource=GLOBAL  ConsistencyAbsTol=0.001  ConsistencyRelTol=0.001  ConsistencyTolFactor=0.001  UseLocalSolver=off  LocalSolverChoice=NE_BACKWARD_EULER_ADVANCER  ResolveIndetEquations=on  FunctionEvalNumThread=1  LocalSolverSampleTime=0.001  DoFixedCost=off  MaxNonlinIter=3  MaxModeIter=2  ComputeImpulses=off  ImpulseIterations=2  LinearAlgebra=auto  LinearAlgebraNumThread=0  EquationFormulation=NE_TIME_EF  DelaysMemoryBudget=1024  AutomaticFiltering=on  FilteringTimeConstant=0.001  PartitionStorageMethod=AS_NEEDED  PartitionMemoryBudget=1024  PartitionMethod=BALANCED  MultibodyUseLocalSolver=off  MultibodyLocalSolverChoice=ODE1  MultibodyLocalSolverSampleTime=0.001
  World : sm_lib/Frames and Transforms/World Frame
  arm_to_world_fixed : sm_lib/Joints/Weld Joint  JointMode=Normal  CompositeWrenchDir=FollowerOnBase  CompositeWrenchFrame=BaseFrame  SenseConstraintForce=off  SenseConstraintTorque=off  SenseTotalForce=off  SenseTotalTorque=off
  panda_joint1 : sm_lib/Joints/Revolute Joint  JointMode=Normal  CompositeWrenchDir=FollowerOnBase  CompositeWrenchFrame=BaseFrame  SenseConstraintForce=off  SenseConstraintTorque=off  SenseTotalForce=off  SenseTotalTorque=off  PositionTargetSpecify=on  PositionTargetPriority=High  PositionTargetValue=q_init(1)  PositionTargetValueUnits=rad  VelocityTargetSpecify=off  VelocityTargetPriority=High  VelocityTargetValue=0  VelocityTargetValueUnits=deg/s  EquilibriumPosition=0  EquilibriumPositionUnits=deg  SpringStiffness=0  SpringStiffnessUnits=N*m/deg  DampingCoefficient=0  DampingCoefficientUnits=kg*m^2/(rad*s)  LowerLimitSpecify=off  LowerLimitBound=-2.8973  LowerLimitBoundUnits=rad  LowerLimitStiffness=1e4  LowerLimitStiffnessUnits=N*m/deg  LowerLimitDamping=10  LowerLimitDampingUnits=N*m/(deg/s)  LowerLimitTransitionRegionWidth=0.1  LowerLimitTransitionRegionWidthUnits=deg  UpperLimitSpecify=off  UpperLimitBound=2.8973  UpperLimitBoundUnits=rad  UpperLimitStiffness=1e4  UpperLimitStiffnessUnits=N*m/deg  UpperLimitDamping=10  UpperLimitDampingUnits=N*m/(deg/s)  UpperLimitTransitionRegionWidth=0.1  UpperLimitTransitionRegionWidthUnits=deg  TorqueActuationMode=InputTorque  MotionActuationMode=ComputedMotion  SensePosition=on  SenseVelocity=on  SenseAcceleration=off  SenseTorqueForce=off  SenseLowerLimitTorqueForce=off  SenseUpperLimitTorqueForce=off
  panda_joint2 : sm_lib/Joints/Revolute Joint  JointMode=Normal  CompositeWrenchDir=FollowerOnBase  CompositeWrenchFrame=BaseFrame  SenseConstraintForce=off  SenseConstraintTorque=off  SenseTotalForce=off  SenseTotalTorque=off  PositionTargetSpecify=on  PositionTargetPriority=High  PositionTargetValue=q_init(2)  PositionTargetValueUnits=rad  VelocityTargetSpecify=off  VelocityTargetPriority=High  VelocityTargetValue=0  VelocityTargetValueUnits=deg/s  EquilibriumPosition=0  EquilibriumPositionUnits=deg  SpringStiffness=0  SpringStiffnessUnits=N*m/deg  DampingCoefficient=0  DampingCoefficientUnits=kg*m^2/(rad*s)  LowerLimitSpecify=off  LowerLimitBound=-1.7628  LowerLimitBoundUnits=rad  LowerLimitStiffness=1e4  LowerLimitStiffnessUnits=N*m/deg  LowerLimitDamping=10  LowerLimitDampingUnits=N*m/(deg/s)  LowerLimitTransitionRegionWidth=0.1  LowerLimitTransitionRegionWidthUnits=deg  UpperLimitSpecify=off  UpperLimitBound=1.7628  UpperLimitBoundUnits=rad  UpperLimitStiffness=1e4  UpperLimitStiffnessUnits=N*m/deg  UpperLimitDamping=10  UpperLimitDampingUnits=N*m/(deg/s)  UpperLimitTransitionRegionWidth=0.1  UpperLimitTransitionRegionWidthUnits=deg  TorqueActuationMode=InputTorque  MotionActuationMode=ComputedMotion  SensePosition=on  SenseVelocity=on  SenseAcceleration=off  SenseTorqueForce=off  SenseLowerLimitTorqueForce=off  SenseUpperLimitTorqueForce=off
  panda_joint3 : sm_lib/Joints/Revolute Joint  JointMode=Normal  CompositeWrenchDir=FollowerOnBase  CompositeWrenchFrame=BaseFrame  SenseConstraintForce=off  SenseConstraintTorque=off  SenseTotalForce=off  SenseTotalTorque=off  PositionTargetSpecify=on  PositionTargetPriority=High  PositionTargetValue=q_init(3)  PositionTargetValueUnits=rad  VelocityTargetSpecify=off  VelocityTargetPriority=High  VelocityTargetValue=0  VelocityTargetValueUnits=deg/s  EquilibriumPosition=0  EquilibriumPositionUnits=deg  SpringStiffness=0  SpringStiffnessUnits=N*m/deg  DampingCoefficient=0  DampingCoefficientUnits=kg*m^2/(rad*s)  LowerLimitSpecify=off  LowerLimitBound=-2.8973  LowerLimitBoundUnits=rad  LowerLimitStiffness=1e4  LowerLimitStiffnessUnits=N*m/deg  LowerLimitDamping=10  LowerLimitDampingUnits=N*m/(deg/s)  LowerLimitTransitionRegionWidth=0.1  LowerLimitTransitionRegionWidthUnits=deg  UpperLimitSpecify=off  UpperLimitBound=2.8973  UpperLimitBoundUnits=rad  UpperLimitStiffness=1e4  UpperLimitStiffnessUnits=N*m/deg  UpperLimitDamping=10  UpperLimitDampingUnits=N*m/(deg/s)  UpperLimitTransitionRegionWidth=0.1  UpperLimitTransitionRegionWidthUnits=deg  TorqueActuationMode=InputTorque  MotionActuationMode=ComputedMotion  SensePosition=on  SenseVelocity=on  SenseAcceleration=off  SenseTorqueForce=off  SenseLowerLimitTorqueForce=off  SenseUpperLimitTorqueForce=off
  panda_joint4 : sm_lib/Joints/Revolute Joint  JointMode=Normal  CompositeWrenchDir=FollowerOnBase  CompositeWrenchFrame=BaseFrame  SenseConstraintForce=off  SenseConstraintTorque=off  SenseTotalForce=off  SenseTotalTorque=off  PositionTargetSpecify=on  PositionTargetPriority=High  PositionTargetValue=q_init(4)  PositionTargetValueUnits=rad  VelocityTargetSpecify=off  VelocityTargetPriority=High  VelocityTargetValue=0  VelocityTargetValueUnits=deg/s  EquilibriumPosition=0  EquilibriumPositionUnits=deg  SpringStiffness=0  SpringStiffnessUnits=N*m/deg  DampingCoefficient=0  DampingCoefficientUnits=kg*m^2/(rad*s)  LowerLimitSpecify=off  LowerLimitBound=-3.0718  LowerLimitBoundUnits=rad  LowerLimitStiffness=1e4  LowerLimitStiffnessUnits=N*m/deg  LowerLimitDamping=10  LowerLimitDampingUnits=N*m/(deg/s)  LowerLimitTransitionRegionWidth=0.1  LowerLimitTransitionRegionWidthUnits=deg  UpperLimitSpecify=off  UpperLimitBound=-0.0698  UpperLimitBoundUnits=rad  UpperLimitStiffness=1e4  UpperLimitStiffnessUnits=N*m/deg  UpperLimitDamping=10  UpperLimitDampingUnits=N*m/(deg/s)  UpperLimitTransitionRegionWidth=0.1  UpperLimitTransitionRegionWidthUnits=deg  TorqueActuationMode=InputTorque  MotionActuationMode=ComputedMotion  SensePosition=on  SenseVelocity=on  SenseAcceleration=off  SenseTorqueForce=off  SenseLowerLimitTorqueForce=off  SenseUpperLimitTorqueForce=off
  panda_joint5 : sm_lib/Joints/Revolute Joint  JointMode=Normal  CompositeWrenchDir=FollowerOnBase  CompositeWrenchFrame=BaseFrame  SenseConstraintForce=off  SenseConstraintTorque=off  SenseTotalForce=off  SenseTotalTorque=off  PositionTargetSpecify=on  PositionTargetPriority=High  PositionTargetValue=q_init(5)  PositionTargetValueUnits=rad  VelocityTargetSpecify=off  VelocityTargetPriority=High  VelocityTargetValue=0  VelocityTargetValueUnits=deg/s  EquilibriumPosition=0  EquilibriumPositionUnits=deg  SpringStiffness=0  SpringStiffnessUnits=N*m/deg  DampingCoefficient=0  DampingCoefficientUnits=kg*m^2/(rad*s)  LowerLimitSpecify=off  LowerLimitBound=-2.8973  LowerLimitBoundUnits=rad  LowerLimitStiffness=1e4  LowerLimitStiffnessUnits=N*m/deg  LowerLimitDamping=10  LowerLimitDampingUnits=N*m/(deg/s)  LowerLimitTransitionRegionWidth=0.1  LowerLimitTransitionRegionWidthUnits=deg  UpperLimitSpecify=off  UpperLimitBound=2.8973  UpperLimitBoundUnits=rad  UpperLimitStiffness=1e4  UpperLimitStiffnessUnits=N*m/deg  UpperLimitDamping=10  UpperLimitDampingUnits=N*m/(deg/s)  UpperLimitTransitionRegionWidth=0.1  UpperLimitTransitionRegionWidthUnits=deg  TorqueActuationMode=InputTorque  MotionActuationMode=ComputedMotion  SensePosition=on  SenseVelocity=on  SenseAcceleration=off  SenseTorqueForce=off  SenseLowerLimitTorqueForce=off  SenseUpperLimitTorqueForce=off
  panda_joint6 : sm_lib/Joints/Revolute Joint  JointMode=Normal  CompositeWrenchDir=FollowerOnBase  CompositeWrenchFrame=BaseFrame  SenseConstraintForce=off  SenseConstraintTorque=off  SenseTotalForce=off  SenseTotalTorque=off  PositionTargetSpecify=on  PositionTargetPriority=High  PositionTargetValue=q_init(6)  PositionTargetValueUnits=rad  VelocityTargetSpecify=off  VelocityTargetPriority=High  VelocityTargetValue=0  VelocityTargetValueUnits=deg/s  EquilibriumPosition=0  EquilibriumPositionUnits=deg  SpringStiffness=0  SpringStiffnessUnits=N*m/deg  DampingCoefficient=0  DampingCoefficientUnits=kg*m^2/(rad*s)  LowerLimitSpecify=off  LowerLimitBound=-0.0175  LowerLimitBoundUnits=rad  LowerLimitStiffness=1e4  LowerLimitStiffnessUnits=N*m/deg  LowerLimitDamping=10  LowerLimitDampingUnits=N*m/(deg/s)  LowerLimitTransitionRegionWidth=0.1  LowerLimitTransitionRegionWidthUnits=deg  UpperLimitSpecify=off  UpperLimitBound=3.7525  UpperLimitBoundUnits=rad  UpperLimitStiffness=1e4  UpperLimitStiffnessUnits=N*m/deg  UpperLimitDamping=10  UpperLimitDampingUnits=N*m/(deg/s)  UpperLimitTransitionRegionWidth=0.1  UpperLimitTransitionRegionWidthUnits=deg  TorqueActuationMode=InputTorque  MotionActuationMode=ComputedMotion  SensePosition=on  SenseVelocity=on  SenseAcceleration=off  SenseTorqueForce=off  SenseLowerLimitTorqueForce=off  SenseUpperLimitTorqueForce=off
  panda_joint7 : sm_lib/Joints/Revolute Joint  JointMode=Normal  CompositeWrenchDir=FollowerOnBase  CompositeWrenchFrame=BaseFrame  SenseConstraintForce=off  SenseConstraintTorque=off  SenseTotalForce=off  SenseTotalTorque=off  PositionTargetSpecify=on  PositionTargetPriority=High  PositionTargetValue=q_init(7)  PositionTargetValueUnits=rad  VelocityTargetSpecify=off  VelocityTargetPriority=High  VelocityTargetValue=0  VelocityTargetValueUnits=deg/s  EquilibriumPosition=0  EquilibriumPositionUnits=deg  SpringStiffness=0  SpringStiffnessUnits=N*m/deg  DampingCoefficient=0  DampingCoefficientUnits=kg*m^2/(rad*s)  LowerLimitSpecify=off  LowerLimitBound=-2.8973  LowerLimitBoundUnits=rad  LowerLimitStiffness=1e4  LowerLimitStiffnessUnits=N*m/deg  LowerLimitDamping=10  LowerLimitDampingUnits=N*m/(deg/s)  LowerLimitTransitionRegionWidth=0.1  LowerLimitTransitionRegionWidthUnits=deg  UpperLimitSpecify=off  UpperLimitBound=2.8973  UpperLimitBoundUnits=rad  UpperLimitStiffness=1e4  UpperLimitStiffnessUnits=N*m/deg  UpperLimitDamping=10  UpperLimitDampingUnits=N*m/(deg/s)  UpperLimitTransitionRegionWidth=0.1  UpperLimitTransitionRegionWidthUnits=deg  TorqueActuationMode=InputTorque  MotionActuationMode=ComputedMotion  SensePosition=on  SenseVelocity=on  SenseAcceleration=off  SenseTorqueForce=off  SenseLowerLimitTorqueForce=off  SenseUpperLimitTorqueForce=off
  panda_joint8 : sm_lib/Joints/Weld Joint  JointMode=Normal  CompositeWrenchDir=FollowerOnBase  CompositeWrenchFrame=BaseFrame  SenseConstraintForce=off  SenseConstraintTorque=off  SenseTotalForce=off  SenseTotalTorque=off
  panda_link0 : Subsystem
  panda_link1 : Subsystem
  panda_link2 : Subsystem
  panda_link3 : Subsystem
  panda_link4 : Subsystem
  panda_link5 : Subsystem
  panda_link6 : Subsystem
  panda_link7 : Subsystem
  panda_link8 : Subsystem
  world : Subsystem
  q : Outport
  q_dot : Outport  Port=2
  wires:
  Demux/6 -> Simulink-PS Converter5/1
  PS-Simulink Converter4/1 -> Mux/5
  PS-Simulink Converter8/1 -> Mux1/2
  tau/1 -> Demux/1
  PS-Simulink Converter11/1 -> Mux1/5
  PS-Simulink Converter2/1 -> Mux/3
  PS-Simulink Converter5/1 -> Mux/6
  Demux/5 -> Simulink-PS Converter4/1
  PS-Simulink Converter7/1 -> Mux1/1
  PS-Simulink Converter3/1 -> Mux/4
  Mux1/1 -> q_dot/1
  Demux/7 -> Simulink-PS Converter6/1
  Demux/4 -> Simulink-PS Converter3/1
  Demux/1 -> Simulink-PS Converter/1
  PS-Simulink Converter10/1 -> Mux1/4
  PS-Simulink Converter/1 -> Mux/1
  PS-Simulink Converter9/1 -> Mux1/3
  Demux/3 -> Simulink-PS Converter2/1
  PS-Simulink Converter6/1 -> Mux/7
  PS-Simulink Converter13/1 -> Mux1/7
  PS-Simulink Converter12/1 -> Mux1/6
  Demux/2 -> Simulink-PS Converter1/1
  PS-Simulink Converter1/1 -> Mux/2
  Mux/1 -> q/1
  connections:
  PS-Simulink Converter8/LConn1 -- panda_joint2/RConn3
  panda_joint8/RConn1 -- panda_link8/LConn1
  panda_joint2/RConn1 -- panda_link2/LConn1
  PS-Simulink Converter11/LConn1 -- panda_joint5/RConn3
  Simulink-PS Converter5/RConn1 -- panda_joint6/LConn2
  Solver Configuration/RConn1 -- world/LConn1 -- MechanismConfiguration/RConn1 -- Rigid Transform/LConn1 -- World/RConn1
  PS-Simulink Converter10/LConn1 -- panda_joint4/RConn3
  panda_joint2/LConn1 -- panda_link1/RConn1
  panda_joint7/RConn2 -- PS-Simulink Converter6/LConn1
  arm_to_world_fixed/RConn1 -- panda_link0/LConn1
  panda_joint6/RConn2 -- PS-Simulink Converter5/LConn1
  PS-Simulink Converter9/LConn1 -- panda_joint3/RConn3
  panda_joint4/RConn1 -- panda_link4/LConn1
  panda_joint7/RConn1 -- panda_link7/LConn1
  panda_joint2/RConn2 -- PS-Simulink Converter1/LConn1
  panda_joint4/RConn2 -- PS-Simulink Converter3/LConn1
  panda_joint4/LConn1 -- panda_link3/RConn1
  PS-Simulink Converter12/LConn1 -- panda_joint6/RConn3
  panda_joint3/RConn2 -- PS-Simulink Converter2/LConn1
  Simulink-PS Converter/RConn1 -- panda_joint1/LConn2
  panda_joint3/LConn1 -- panda_link2/RConn1
  panda_joint1/RConn1 -- panda_link1/LConn1
  panda_joint3/RConn1 -- panda_link3/LConn1
  PS-Simulink Converter7/LConn1 -- panda_joint1/RConn3
  panda_joint1/RConn2 -- PS-Simulink Converter/LConn1
  panda_joint1/LConn1 -- panda_link0/RConn1
  panda_joint5/RConn1 -- panda_link5/LConn1
  panda_joint6/RConn1 -- panda_link6/LConn1
  Simulink-PS Converter1/RConn1 -- panda_joint2/LConn2
  Simulink-PS Converter6/RConn1 -- panda_joint7/LConn2
  arm_to_world_fixed/LConn1 -- world/RConn1
  panda_joint7/LConn1 -- panda_link6/RConn1
  panda_joint5/LConn1 -- panda_link4/RConn1
  panda_joint8/LConn1 -- panda_link7/RConn1
  PS-Simulink Converter13/LConn1 -- panda_joint7/RConn3
  Simulink-PS Converter4/RConn1 -- panda_joint5/LConn2
  Simulink-PS Converter2/RConn1 -- panda_joint3/LConn2
  panda_joint6/LConn1 -- panda_link5/RConn1
  Simulink-PS Converter3/RConn1 -- panda_joint4/LConn2
  panda_joint5/RConn2 -- PS-Simulink Converter4/LConn1
  Rigid Transform1/RConn1 -- Cylindrical Solid/RConn1
  Rigid Transform1/LConn1 -- Rigid Transform/RConn1
